simulink model "EMT_ML.before_diagnostic_fixes"  (R2024b)
settings: Solver=ode5  StartTime=0.0  StopTime=200  FixedStep=0.002  RelTol=1e-3
model workspace (MAT data in the model file):
  A = 7.3
  B = 2.71
  C0_shift = 200
  C1_shift = 200
  C2_shift = 200
  Cb = 70
  Cd = 0.6
  EMSInputBus : Simulink.Bus (value not decoded)
  Fb_max = 247500
  JA = 0.4
  JB = 0.4
  JZ = 0.4
  Jc1r2 = 0.01
  Jc3r4 = 0.01
  Jc4 = 0.01
  Je = 2.5
  Jh = 0.01
  Jq1 = 0.01
  Jq2 = 0.01
  Jr1 = 0.01
  Jr3s4 = 0.01
  Js123 = 0.01
  L = 4.472
  NE = [1600 1600 1600 1600 1600 1600 1600 1600 1600 1600 1600 1600 ... (840 elements, 30x28)]
  N_Te = 30
  N_ne = 28
  PE = [0 100.366530527 133.710336161 167.221698607 195.706356687 221.845219395 250.497434286 278.144308305 305.288511886 330.086920096 352.87464656 374.489475338 ... (840 elements, 30x28)]
  PN0 = 0
  Pb_epr = [-45 -45 -40 -30 0 30 40 45 45]
  Pb_max = [0 40 45 45 45]
  Pb_min = [-45 -45 -45 -40 0]
  Pe_ass = 230
  Pe_max = 1103
  Peg = [0 100 120 140 160 180 200 220 240 260 280 300 ... (53 elements, 1x53)]
  R_map = [0.09 0.089 0.09 0.091 0.092 0.093 0.094 0.095 0.096 0.097 0.098]
  SF_C0 = 1.5
  SF_C1 = 1.5
  SF_C2 = 1.5
  SF_Z1 = 1.5
  SF_Z2 = 1.5
  SF_ZD = 1.5
  SOC0 = 60
  SOC_epr = [30 31 50 59 60 61 70 79 80]
  SOC_map = [0 10 20 30 40 50 60 70 80 90 100]
  TA_max_map = [588.855 593.803361345 598.83559322 603.953846154 609.160344828 614.457391304 619.847368421 625.332743363 630.916071429 636.6 642.387272727 648.280733945 ... (115 elements, 1x115)]
  TA_min_map = [-588.855 -593.803361345 -598.83559322 -603.953846154 -609.160344828 -614.457391304 -619.847368421 -625.332743363 -630.916071429 -636.6 -642.387272727 -648.280733945 ... (115 elements, 1x115)]
  TAf = 0
  TB_max_map = [588.855 593.803361345 598.83559322 603.953846154 609.160344828 614.457391304 619.847368421 625.332743363 630.916071429 636.6 642.387272727 648.280733945 ... (115 elements, 1x115)]
  TB_min_map = [-588.855 -593.803361345 -598.83559322 -603.953846154 -609.160344828 -614.457391304 -619.847368421 -625.332743363 -630.916071429 -636.6 -642.387272727 -648.280733945 ... (115 elements, 1x115)]
  TBf = 0
  TE = [0 599 798 998 1168 1324 1495 1660 1822 1970 2106 2235 ... (840 elements, 30x28)]
  TS_A = 0.2
  TS_B = 0.2
  TS_C0 = 0.2
  TS_C1 = 0.2
  TS_C2 = 0.2
  TS_Z = 0.2
  TS_Z1 = 0.2
  TS_Z2 = 0.2
  TS_ZD = 0.2
  TZ_max_map = [537.13125 540.509433962 543.930379747 547.394904459 550.903846154 554.458064516 558.058441558 561.705882353 565.401315789 569.145695364 572.94 576.785234899 ... (131 elements, 1x131)]
  TZ_min_map = [-537.13125 -540.509433962 -543.930379747 -547.394904459 -550.903846154 -554.458064516 -558.058441558 -561.705882353 -565.401315789 -569.145695364 -572.94 -576.785234899 ... (131 elements, 1x131)]
  TZf = 0
  T_generator = [0 185 493.333333333 801.666666667 1110 1418.33333333 1726.66666667]
  T_motor = [0 185 493.333333333 801.666666667 1110 1418.33333333 1726.66666667]
  Te_map = [0 599 798 998 1168 1324 1495 1660 1822 1970 2106 2235 ... (30 elements, 1x30)]
  Te_max = 2754
  Te_max_map = [1168 1324 1495 1660 1822 1970 2106 2235 2355 2458 2543 2606 ... (28 elements, 1x28)]
  Te_start = 1600
  Tef = 100
  Teg = [0 596.8125 636.6 718.741935484 799.916230366 859.41 954.422788606 954.9 996.417391304 1078.98305085 1114.05 1169.26530612 ... (53 elements, 1x53)]
  Temax = 998
  Time = [0 0.1 0.2 0.3 0.4 0.5 0.6 0.7 0.8 0.9 1 1.1 ... (2001 elements, 1x2001)]
  Time_ele = [0 4 8 12 16 20 24 28 32 36 40 44 ... (401 elements, 1x401)]
  Time_fg = [0 2 4 6 8 10 12 14 16 18 20 22 ... (801 elements, 1x801)]
  Tmax_C0 = 2754
  Tmax_C1 = 3505.25455609
  Tmax_C2 = 3505.25455609
  Tmax_Z1 = 5584.80955498
  Tmax_Z2 = 16307.6439005
  Tmax_ZD = 3855.6
  Ts_e = 0.1
  Uoc_map = [814.5 917 933.25 945.75 958.25 969.25 978 985.25 993.25 1003.25 1050]
  V_Shift12 = 32
  V_Shift21 = 25
  V_Start = 10
  Voltage0 = 900
  Voltage_epr = [750 760 900 1000 1050]
  Y_engine = 0.955
  Yc = 0.98
  Yh = 0.96
  Yo = 0.92
  Yq = 0.94
  Z1_shift = 200
  Z2_shift = 200
  a11 = 1.54241568346
  a11_L = 1.54241568346
  a12 = -3.86074191629
  a12_L = 2.43173643789
  a21 = -1.04963112005
  a22 = 2.46948356808
  b11 = 0
  b11_L = 0
  b12 = 3.33
  b12_L = 7.8036
  b21 = 2.23571428571
  b22 = -2.13
  c11 = -0.648333656565
  c12 = 0
  c21 = -0.648333656565
  c22 = 0.680511182109
  controller_id = 1
  controller_name = 'Existing heuristic-grid EMS'
  cycle_grade = [0 0 0 0 0 0 0 0 0 0 0 0 ... (2001 elements, 1x2001)]
  cycle_road = [0.045 0.045 0.045 0.045 0.045 0.045 0.045 0.045 0.045 0.045 0.045 0.045 ... (2001 elements, 1x2001)]
  cycle_steering = [0 0 0 0 0 0 0 0 0 0 0 0 ... (2001 elements, 1x2001)]
  cycle_time = [0 0.1 0.2 0.3 0.4 0.5 0.6 0.7 0.8 0.9 1 1.1 ... (2001 elements, 1x2001)]
  d11 = -0.751666343435
  d12 = 0.3003003003
  d21 = -0.751666343435
  d22 = 0.319488817891
  e11 = -1.54241568346
  e12 = 0
  e21 = 1.04963112005
  e22 = -2.23571428571
  eff_generator = [0.8 0.8 0.79 0.79 0.76 0.74 0.72 0.8 0.85 0.88 0.85 0.8 ... (84 elements, 7x12)]
  eff_motor = [0.8 0.8 0.79 0.79 0.76 0.74 0.72 0.8 0.85 0.88 0.85 0.8 ... (84 elements, 7x12)]
  ele_map = [10 11.46 14.13 19.24 20.94 23.21 20.29 20.23 22.28 17.66 16.24 18.95 ... (401 elements, 1x401)]
  ems_runtime_config : object (value not decoded)
  f11 = -3.86074191629
  f12 = 3.33
  f21 = 2.46948356808
  f22 = -2.13
  fg = 0.045
  fg_map = [0.0125 0.0215 0.0332 0.0452 0.0525 0.0589 0.0584 0.0592 0.0621 0.0576 0.055 0.0572 ... (801 elements, 1x801)]
  fuel_gpkwh = [269.874826377 269.874826377 260.084605263 254.895150301 249.802821062 244.062054381 234.972466555 226.630558735 223.93243551 227.612775381 231.379615385 228.983738255 ... (840 elements, 30x28)]
  fuel_map = [269.874826377 269.874826377 260.084605263 254.895150301 249.802821062 244.062054381 234.972466555 226.630558735 223.93243551 227.612775381 231.379615385 228.983738255 ... (840 elements, 30x28)]
  fuel_map_N = [269.874826377 269.874826377 260.084605263 254.895150301 249.802821062 nan nan nan nan nan nan nan ... (840 elements, 30x28)]
  i = 28
  ic = 4.42
  iq = 1.4
  it = 4
  j = 30
  k1 = 2.13
  k2 = 2.13
  k3 = 2.33
  k4 = 1.92
  kh = 2.88
  kq = 2.17
  kt = 1.83
  mass = 45000
  miu_max = 0.8
  nA_map = [-6000 -5950 -5900 -5850 -5800 -5750 -5700 -5650 -5600 -5550 -5500 -5450 ... (115 elements, 1x115)]
  nA_max = 6000
  nA_min = -6000
  nB_map = [-6000 -5950 -5900 -5850 -5800 -5750 -5700 -5650 -5600 -5550 -5500 -5450 ... (115 elements, 1x115)]
  nB_max = 6000
  nB_min = -6000
  nB_start = 0
  nZ_map = [-8000 -7950 -7900 -7850 -7800 -7750 -7700 -7650 -7600 -7550 -7500 -7450 ... (131 elements, 1x131)]
  nZ_max = 8000
  nZ_min = -8000
  n_generator = [0 318.5 796.25 1274 1751.75 2229.5 2707.25 3185 3662.75 4140.5 4618.25 7007]
  n_motor = [0 318.5 796.25 1274 1751.75 2229.5 2707.25 3185 3662.75 4140.5 4618.25 7007]
  ne_idl = 3000
  ne_map = [1600 1700 1800 1900 2000 2100 2200 2300 2400 2500 2600 2700 ... (28 elements, 1x28)]
  ne_max = 4200
  ne_min = 1600
  ne_start = 200
  neg = [1600 1600 1800 1860 1910 2000 2001 2200 2300 2301 2400 2450 ... (53 elements, 1x53)]
  no_Shift12 = 1589.43589002
  no_Shift21 = 1241.74678908
  rz = 0.318
  startup_feedback_delay_s = 0.002
  startup_power_share = 0.5
  startup_speed_regularizer_rpm = 100
  v_cyc = [0 0 0 0 0 0 0 0 0 0 0 0 ... (2001 elements, 1x2001)]
  voltage_HighA = 1050
  voltage_HighB = 1050
  voltage_HighZ = 1050
  voltage_LowA = 750
  voltage_LowB = 750
  voltage_LowZ = 750
symbols that are objects in the model workspace (value not decoded): ems_runtime_config
undefined symbols (not defined in the file or in its folder): sigbuilder_block
libraries: fl_lib x82, nesl_utility x55, simulink x49, sdl_lib x10, simulink_need_slupdate x6, powerlib_extras x1
(part 4 of 7)

== system EMT_ML.before_diagnostic_fixes/Control Unit/Control/Power Distribution/Electric Power Requirement ==
  Voltage : Inport
  SOC : Inport  Port=2
  ElectricPower : Inport  Port=3
  1-D Lookup Table : Lookup_n-D  NumberOfTableDimensions=1  BreakpointsForDimension1=SOC_epr  Table=Pb_epr  RndMeth=Simplest
  1-D Lookup Table2 : Lookup_n-D  NumberOfTableDimensions=1  BreakpointsForDimension1=Voltage_epr  Table=Pb_max  RndMeth=Simplest
  1-D Lookup Table3 : Lookup_n-D  NumberOfTableDimensions=1  BreakpointsForDimension1=Voltage_epr  Table=Pb_min  RndMeth=Simplest
  Add : Sum  Inputs=+--
  Constant : Constant  Value=PN0
  Data : Subsystem
  Memory3 : Memory  InitialCondition=SOC0
  Memory7 : Memory  InitialCondition=SOC0
  Mux : Mux
  PZ_com : Constant  Value=0
  Saturation1 : Saturate  UpperLimit=max(SOC_epr)  LowerLimit=min(SOC_epr)
  Saturation2 : Saturate  UpperLimit=max(Voltage_epr)  LowerLimit=min(Voltage_epr)
  PN_k : Outport
  wires:
  1-D Lookup Table2/1 -> Data/2(PN_max), Mux/2
  1-D Lookup Table3/1 -> Data/3(PN_min), Mux/3
  Saturation2/1 -> 1-D Lookup Table3/1, 1-D Lookup Table2/1
  Voltage/1 -> Memory7/1
  Saturation1/1 -> 1-D Lookup Table/1
  Add/1 -> Data/1(PN_com), Mux/1
  1-D Lookup Table/1 -> Add/1
  Memory3/1 -> Saturation1/1
  SOC/1 -> Memory3/1
  Mux/1 -> PN_k/1
  Memory7/1 -> Saturation2/1
  Constant/1 -> Add/3
  ElectricPower/1 -> Add/2
  PZ_com/1 -> Mux/4

== system EMT_ML.before_diagnostic_fixes/Control Unit/Control/Power Distribution/Feasible Control Range ==
  stage : Inport
  ne_act : Inport  Port=2
  v_act : Inport  Port=3
  Memory1 : Memory
  Memory5 : Memory
  State Calculation : Subsystem
  State Predition : Subsystem
  stage_k : Outport
  ne_k : Outport  Port=2
  no_k : Outport  Port=3
  Te_k : Outport  Port=4
  TA_k : Outport  Port=5
  TB_k : Outport  Port=6
  wires:
  State Predition/3(no_k) -> no_k/1
  State Predition/4(Te_k) -> Te_k/1
  State Predition/5(TA_k) -> TA_k/1
  State Predition/6(TB_k) -> TB_k/1
  State Predition/2(ne_k) -> ne_k/1
  State Predition/1(stage_k) -> stage_k/1
  ne_act/1 -> Memory5/1
  stage/1 -> State Calculation/1(s)
  v_act/1 -> Memory1/1
  Memory5/1 -> State Calculation/2(ne)
  Memory1/1 -> State Calculation/3(v_act)
  State Calculation/1(stage) -> State Predition/1(stage)
  State Calculation/2(ne_act) -> State Predition/2(ne_act)
  State Calculation/3(nA_act) -> State Predition/3(nA_act)
  State Calculation/4(nB_act) -> State Predition/4(nB_act)
  State Calculation/5(no_act) -> State Predition/5(no_act)

== system EMT_ML.before_diagnostic_fixes/Control Unit/Control/Power Distribution/Oil Control ==
  Demux : Demux
      settings: DisplayOption=none
  Transfer Fcn1 : TransferFcn  Denominator=[TS_C0 1]
  Transfer Fcn2 : TransferFcn  Denominator=[TS_Z1 1]
  Transfer Fcn3 : TransferFcn  Denominator=[TS_Z2 1]
  Transfer Fcn4 : TransferFcn  Denominator=[TS_C1 1]
  tag scope: Press_C0=global, Press_C1=global, Press_Z1=global, Press_Z2=global
  wires:
  Transfer Fcn1/1 -> [Press_C0]
  Transfer Fcn2/1 -> [Press_Z1]
  Demux/1 -> Transfer Fcn1/1
  Demux/4 -> Transfer Fcn4/1
  Demux/3 -> Transfer Fcn3/1
  Demux/2 -> Transfer Fcn2/1
  Transfer Fcn4/1 -> [Press_C1]
  Transfer Fcn3/1 -> [Press_Z2]
  [Press] -> Demux/1

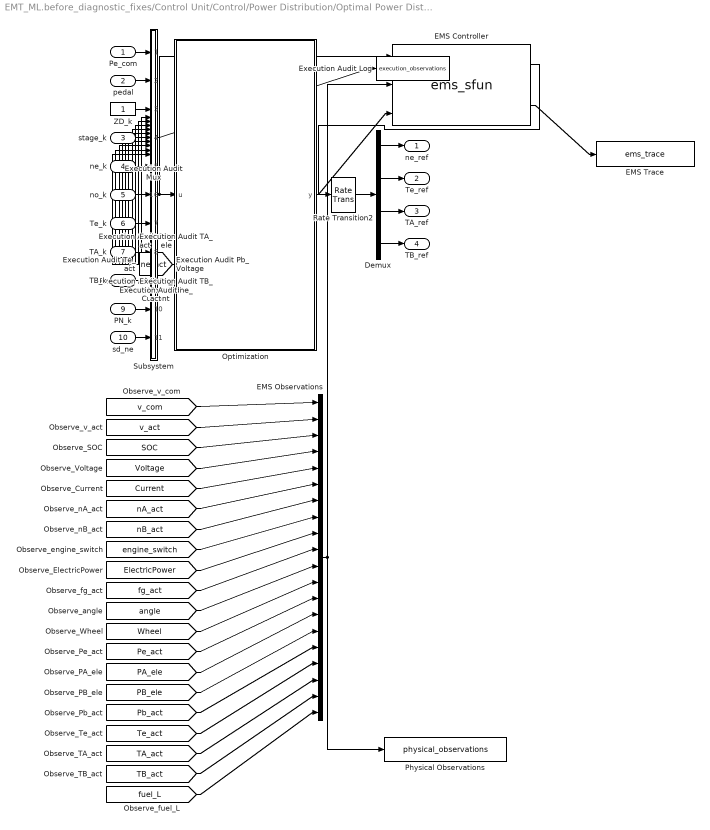
== system EMT_ML.before_diagnostic_fixes/Control Unit/Control/Power Distribution/Optimal Power Distribution ==
  Pe_com : Inport
  pedal : Inport  Port=2
  stage_k : Inport  Port=3
  ne_k : Inport  Port=4
  no_k : Inport  Port=5
  Te_k : Inport  Port=6
  TA_k : Inport  Port=7
  TB_k : Inport  Port=8
  PN_k : Inport  Port=9
  sd_ne : Inport  Port=10
  Demux : Demux
  EMS Controller : M-S-Function  FunctionName=ems_sfun  Parameters=ems_runtime_config,controller_id
  EMS Observations : Mux  Inputs=20
  EMS Trace : ToWorkspace  VariableName=ems_trace  SaveFormat=Structure With Time  SampleTime=0.02
  Execution Audit Log : ToWorkspace  VariableName=execution_observations  SaveFormat=Structure With Time  SampleTime=0.002
  Execution Audit Mux : Mux  Inputs=10
  "Optimization " : MATLAB Function  TreatAsAtomicUnit=on  SystemSampleTime=0.02
  Physical Observations : ToWorkspace  VariableName=physical_observations  SaveFormat=Structure With Time  SampleTime=0.002
  Rate Transition2 : RateTransition
  Subsystem : Subsystem  mask{Parameter1=on}
      mask prompts: Parameter1 "11"
  ZD_k : Constant
  ne_ref : Outport
  Te_ref : Outport  Port=2
  TA_ref : Outport  Port=3
  TB_ref : Outport  Port=4
  wires:
  Demux/1 -> ne_ref/1
  pedal/1 -> Subsystem/2(In2)
  Pe_com/1 -> Subsystem/1(In1)
  ZD_k/1 -> Subsystem/3(In3)
  ne_k/1 -> Subsystem/5(In5)
  no_k/1 -> Subsystem/6(In6)
  Te_k/1 -> Subsystem/7(In7)
  TA_k/1 -> Subsystem/8(In8)
  TB_k/1 -> Subsystem/9(In9)
  PN_k/1 -> Subsystem/10(In10)
  Demux/4 -> TB_ref/1
  Demux/3 -> TA_ref/1
  Demux/2 -> Te_ref/1
  Subsystem/1(Out) -> "Optimization "/1(u), EMS Controller/1
  stage_k/1 -> Subsystem/4(In4)
  Rate Transition2/1 -> Demux/1
  sd_ne/1 -> Subsystem/11(In11)
  [v_com] -> EMS Observations/1
  [v_act] -> EMS Observations/2
  [SOC] -> EMS Observations/3
  [Voltage] -> EMS Observations/4
  [Current] -> EMS Observations/5
  [nA_act] -> EMS Observations/6
  [nB_act] -> EMS Observations/7
  [engine_switch] -> EMS Observations/8
  [ElectricPower] -> EMS Observations/9
  [fg_act] -> EMS Observations/10
  [angle] -> EMS Observations/11
  [Wheel] -> EMS Observations/12
  [Pe_act] -> EMS Observations/13
  [PA_ele] -> EMS Observations/14
  [PB_ele] -> EMS Observations/15
  [Pb_act] -> EMS Observations/16
  [Te_act] -> EMS Observations/17
  [TA_act] -> EMS Observations/18
  [TB_act] -> EMS Observations/19
  [fuel_L] -> EMS Observations/20
  EMS Observations/1 -> EMS Controller/2, Physical Observations/1
  "Optimization "/1(y) -> EMS Controller/3
  EMS Controller/1 -> Rate Transition2/1
  EMS Controller/2 -> EMS Trace/1
  [ne_act] -> Execution Audit Mux/1
  [Te_act] -> Execution Audit Mux/2
  [Pe_act] -> Execution Audit Mux/3
  [TA_act] -> Execution Audit Mux/4
  [TB_act] -> Execution Audit Mux/5
  [PA_ele] -> Execution Audit Mux/6
  [PB_ele] -> Execution Audit Mux/7
  [Pb_act] -> Execution Audit Mux/8
  [Current] -> Execution Audit Mux/9
  [Voltage] -> Execution Audit Mux/10
  Execution Audit Mux/1 -> Execution Audit Log/1

== system EMT_ML.before_diagnostic_fixes/Control Unit/Control/Power Distribution/Pedal Interpretation ==
  Pedal : Inport
  Brake Control : Subsystem
  Data : Subsystem
  Engine Power Requirement : Subsystem
  Subsystem7 : Subsystem
  Subsystem8 : Subsystem
  Fb_ref : Outport
  Pe_com : Outport  Port=2
  wires:
  Engine Power Requirement/1(Pe_com) -> Pe_com/1, Data/3(Pe_com)
  Pedal/1 -> Subsystem7/1(0), Subsystem8/1(0)
  Subsystem7/1(1) -> Engine Power Requirement/1(Acc_pedal), Data/2(Acc_pedal)
  Subsystem8/1(1) -> Brake Control/1(Dec_pedal), Data/1(Dec_pedal)
  Brake Control/1(Fb_ref) -> Fb_ref/1

== system EMT_ML.before_diagnostic_fixes/Control Unit/Control/Power Distribution/Subsystem ==
  Discrete PID Controller : powerlib_extras/Discrete  Control Blocks/Discrete PID Controller  Kp=0.5  Ki=0.1  Kd=0  TcD=1  Par_Limits=[200 -200]  Init=0  Ts=0.5
  Sum : Sum  Inputs=|+-
  sd_ne : Outport
  wires:
  [ne_act] -> Sum/2
  Sum/1 -> Discrete PID Controller/1
  Discrete PID Controller/1 -> sd_ne/1
  [ne_ref] -> Sum/1

== system EMT_ML.before_diagnostic_fixes/Control Unit/Control/Prepare Stage/brack force ==
  Constant1 : Constant  Value=Fb_max
  Fb_com : Outport
  wires:
  Constant1/1 -> Fb_com/1

== system EMT_ML.before_diagnostic_fixes/Control Unit/Control/Prepare Stage/clutches condition ==
  Mux1 : Mux
  Subsystem : Subsystem
  Subsystem1 : Subsystem
  Subsystem2 : Subsystem
  Subsystem3 : Subsystem
  clutch_com : Outport
  wires:
  Subsystem/1(C0) -> Mux1/1
  Subsystem2/1(C1) -> Mux1/4
  Subsystem1/1(Z2) -> Mux1/3
  Subsystem3/1(Z1) -> Mux1/2
  Mux1/1 -> clutch_com/1

== system EMT_ML.before_diagnostic_fixes/Control Unit/Control/Prepare Stage/engine swich ==
  Compare To Constant2 : simulink/Logic and Bit Operations/Compare To Constant  relop=>  const=ne_start  OutDataTypeStr=uint8
  Constant : Constant
  Memory2 : Memory
  Triggered Subsystem : Subsystem  TreatAsAtomicUnit=on
  engine_swich : Outport
  wires:
  Triggered Subsystem/1(Out1) -> engine_swich/1
  Constant/1 -> Triggered Subsystem/1(In1)
  Memory2/1 -> Compare To Constant2/1
  [ne_act] -> Memory2/1
  Compare To Constant2/1 -> Triggered Subsystem/Trigger

== system EMT_ML.before_diagnostic_fixes/Control Unit/Control/Prepare Stage/engine torque ==
  Subsystem1 : Subsystem
  Te_com : Outport
  wires:
  Subsystem1/1(Te_com) -> Te_com/1
  [ne_act] -> Subsystem1/1(ne_act)

== system EMT_ML.before_diagnostic_fixes/Control Unit/Control/Prepare Stage/motorA torque ==
  Constant2 : Constant  Value=0
  Subsystem : Subsystem
  Switch : Switch  Criteria=u2 > Threshold  Threshold=0.1  SaturateOnIntegerOverflow=off  InputSameDT=off
  TA_com1 : Subsystem
  TA_com : Outport
  wires:
  Switch/1 -> TA_com/1
  Subsystem/1(Judge) -> Switch/2
  Constant2/1 -> Switch/3
  TA_com1/1(TA_com) -> Switch/1

== system EMT_ML.before_diagnostic_fixes/Control Unit/Control/Prepare Stage/motorB torque ==
  Lookup Table : Lookup  InputValues=nB_map  Table=TB_max_map*1.5  SaturateOnIntegerOverflow=off
  Lookup Table1 : Lookup  InputValues=nB_map  Table=TB_min_map*1.5  SaturateOnIntegerOverflow=off
  Saturation Dynamic : simulink/Discontinuities/Saturation Dynamic  OutMin=[]  OutMax=[]  OutDataTypeStr=Inherit: Same as second input  OutDataType=sfix(16)  OutScaling=2^-10  DoSatur=off
  Saturation1 : Saturate  UpperLimit=max(nB_map)  LowerLimit=min(nB_map)
  Saturation2 : Saturate  UpperLimit=max(nB_map)  LowerLimit=min(nB_map)
  Subsystem1 : Subsystem
  TB_com : Outport
  wires:
  Saturation Dynamic/1 -> TB_com/1
  [nB_act] -> Subsystem1/1(nB_act), Saturation1/1, Saturation2/1
  Lookup Table/1 -> Saturation Dynamic/1
  Lookup Table1/1 -> Saturation Dynamic/3
  Saturation1/1 -> Lookup Table/1
  Saturation2/1 -> Lookup Table1/1
  Subsystem1/1(TB_com) -> Saturation Dynamic/2

== system EMT_ML.before_diagnostic_fixes/Control Unit/Control/Prepare Stage/motorZ torque ==
  Lookup Table : Lookup  InputValues=nZ_map  Table=TZ_max_map  SaturateOnIntegerOverflow=off
  Lookup Table1 : Lookup  InputValues=nZ_map  Table=TZ_min_map  SaturateOnIntegerOverflow=off
  Saturation Dynamic : simulink/Discontinuities/Saturation Dynamic  OutMin=[]  OutMax=[]  OutDataTypeStr=Inherit: Same as second input  OutDataType=sfix(16)  OutScaling=2^-10  DoSatur=off
  Saturation1 : Saturate  UpperLimit=max(nZ_map)  LowerLimit=min(nZ_map)
  Saturation2 : Saturate  UpperLimit=max(nZ_map)  LowerLimit=min(nZ_map)
  Subsystem1 : Subsystem
  TZ_com : Outport
  wires:
  Saturation Dynamic/1 -> TZ_com/1
  [nZ_act] -> Saturation1/1, Saturation2/1, Subsystem1/1(nZ_act)
  Lookup Table/1 -> Saturation Dynamic/1
  Lookup Table1/1 -> Saturation Dynamic/3
  Saturation1/1 -> Lookup Table/1
  Saturation2/1 -> Lookup Table1/1
  Subsystem1/1(TZ_com) -> Saturation Dynamic/2

== system EMT_ML.before_diagnostic_fixes/Control Unit/Control/Shift Stage/EVT1->EVT2 ==
  Mux : Mux  Inputs=7
  brack force : Subsystem
  clutches condition : Subsystem
  engine swich : Subsystem
  engine torque : Subsystem
  motorA torque : Subsystem
  motorB torque : Subsystem
  motorZ torque : Subsystem
  control : Outport
  wires:
  motorB torque/1(TB_com) -> Mux/5
  motorA torque/1(TA_com) -> Mux/4
  engine torque/1(Te_com) -> Mux/3
  Mux/1 -> control/1
  engine swich/1(engine_swich) -> Mux/2
  clutches condition/1(clutch_com) -> Mux/1
  brack force/1(Fb_com) -> Mux/7
  motorZ torque/1(TZ_com) -> Mux/6

== system EMT_ML.before_diagnostic_fixes/Control Unit/Control/Shift Stage/EVT2->EVT1 ==
  Mux : Mux  Inputs=7
  brack force : Subsystem
  clutches condition : Subsystem
  engine swich : Subsystem
  engine torque : Subsystem
  motorA torque : Subsystem
  motorB torque : Subsystem
  motorZ torque : Subsystem
  control : Outport
  wires:
  motorB torque/1(TB_com) -> Mux/5
  motorA torque/1(TA_com) -> Mux/4
  Mux/1 -> control/1
  engine torque/1(Te_com) -> Mux/3
  engine swich/1(engine_swich) -> Mux/2
  clutches condition/1(clutch_com) -> Mux/1
  brack force/1(Fb_com) -> Mux/7
  motorZ torque/1(TZ_com) -> Mux/6

== system EMT_ML.before_diagnostic_fixes/Control Unit/Control/Shift Stage/Shift Judge ==
  1 : Constant
  Add : Sum
  Compare To Constant1 : simulink/Logic and Bit Operations/Compare To Constant  relop=>  const=1  OutDataTypeStr=uint8
  Data Type Conversion1 : DataTypeConversion  SaturateOnIntegerOverflow=off  RndMeth=Floor
  Fcn : Fcn  Expr=V_Shift21+5*u
  Logical Operator1 : Logic  AllPortsSameDT=off  OutDataTypeStr=boolean
  Memory1 : Memory
  Memory2 : Memory
  Memory5 : Memory
  Relational Operator : RelationalOperator  Operator=<=  OutDataTypeStr=boolean  InputSameDT=off
  shift : Outport
  wires:
  Data Type Conversion1/1 -> Add/2
  Fcn/1 -> Relational Operator/2
  Memory1/1 -> Fcn/1
  [Acc_pedal] -> Memory1/1
  Logical Operator1/1 -> Data Type Conversion1/1
  Compare To Constant1/1 -> Logical Operator1/2
  Relational Operator/1 -> Logical Operator1/1
  [v_act] -> Memory2/1
  Memory2/1 -> Relational Operator/1
  [stage] -> Memory5/1
  Memory5/1 -> Compare To Constant1/1
  1/1 -> Add/1
  Add/1 -> shift/1

== system EMT_ML.before_diagnostic_fixes/Control Unit/Control/Stage Judge/EVT1_H Stage ==
  Compare To Constant1 : simulink/Logic and Bit Operations/Compare To Constant  relop=>  const=0.9  OutDataTypeStr=uint8
  Compare To Constant6 : simulink/Logic and Bit Operations/Compare To Constant  relop=>=  const=0.9  OutDataTypeStr=uint8
  Data Type Conversion : DataTypeConversion  SaturateOnIntegerOverflow=off  RndMeth=Floor
  Logical Operator1 : Logic  AllPortsSameDT=off  OutDataTypeStr=boolean
  Memory1 : Memory
  Memory6 : Memory
  Out1 : Outport
  wires:
  Data Type Conversion/1 -> Out1/1
  Logical Operator1/1 -> Data Type Conversion/1
  Memory1/1 -> Compare To Constant1/1
  [Press_C0] -> Memory1/1
  [Press_Z2] -> Memory6/1
  Memory6/1 -> Compare To Constant6/1
  Compare To Constant1/1 -> Logical Operator1/1
  Compare To Constant6/1 -> Logical Operator1/2

== system EMT_ML.before_diagnostic_fixes/Control Unit/Control/Stage Judge/EVT2 Stage ==
  Add : Sum
  Compare To Constant10 : simulink/Logic and Bit Operations/Compare To Constant  relop=>=  const=2  OutDataTypeStr=uint8
  Compare To Constant11 : simulink/Logic and Bit Operations/Compare To Constant  relop=>  const=0.1  OutDataTypeStr=uint8
  Compare To Constant2 : simulink/Logic and Bit Operations/Compare To Constant  relop=<  const=0.9  OutDataTypeStr=uint8
  Compare To Constant3 : simulink/Logic and Bit Operations/Compare To Constant  relop=<=  const=0.1  OutDataTypeStr=uint8
  Compare To Constant4 : simulink/Logic and Bit Operations/Compare To Constant  relop=>=  const=0.9  OutDataTypeStr=uint8
  Data Type Conversion : DataTypeConversion  SaturateOnIntegerOverflow=off  RndMeth=Floor
  Gain : Gain  Gain=3
  Gain1 : Gain  Gain=2
  Logical Operator : Logic  AllPortsSameDT=off  OutDataTypeStr=boolean
  Logical Operator4 : Logic  Inputs=3  AllPortsSameDT=off  OutDataTypeStr=boolean
  Memory{2..4,10..11} (5 alike) : Memory
  Out1 : Outport
  wires:
  Gain1/1 -> Add/1
  Data Type Conversion/1 -> Out1/1
  Add/1 -> Data Type Conversion/1
  Logical Operator4/1 -> Gain1/1
  Gain/1 -> Add/2
  [Press_Z2] -> Memory3/1
  Memory3/1 -> Compare To Constant3/1
  [Press_C1] -> Memory4/1
  Memory4/1 -> Compare To Constant4/1
  Compare To Constant3/1 -> Logical Operator/1
  Compare To Constant4/1 -> Logical Operator/2
  Logical Operator/1 -> Gain/1
  Compare To Constant2/1 -> Logical Operator4/2
  [Press_Z2] -> Memory2/1
  Memory2/1 -> Compare To Constant2/1
  [stage] -> Memory10/1
  Memory10/1 -> Compare To Constant10/1
  Compare To Constant10/1 -> Logical Operator4/1
  [Press_Z2] -> Memory11/1
  Memory11/1 -> Compare To Constant11/1
  Compare To Constant11/1 -> Logical Operator4/3

== system EMT_ML.before_diagnostic_fixes/Control Unit/Control/Stage Judge/Prepare Stage ==
  Constant2 : Constant  Value=0
  Out1 : Outport
  wires:
  Constant2/1 -> Out1/1

== system EMT_ML.before_diagnostic_fixes/Control Unit/Control/Stage Judge/Shift Stage ==
  Compare To Constant5 : simulink/Logic and Bit Operations/Compare To Constant  relop=>  const=0.1  OutDataTypeStr=uint8
  Compare To Constant9 : simulink/Logic and Bit Operations/Compare To Constant  relop=>  const=0.1  OutDataTypeStr=uint8
  Data Type Conversion : DataTypeConversion  SaturateOnIntegerOverflow=off  RndMeth=Floor
  Logical Operator2 : Logic  AllPortsSameDT=off  OutDataTypeStr=boolean
  Memory5 : Memory
  Memory9 : Memory
  Out1 : Outport
  wires:
  Data Type Conversion/1 -> Out1/1
  Logical Operator2/1 -> Data Type Conversion/1
  Compare To Constant5/1 -> Logical Operator2/2
  [Press_C1] -> Memory5/1
  Memory5/1 -> Compare To Constant5/1
  [Press_Z2] -> Memory9/1
  Memory9/1 -> Compare To Constant9/1
  Compare To Constant9/1 -> Logical Operator2/1

== system EMT_ML.before_diagnostic_fixes/Control Unit/Driver/Electric Power Requirement/Subsystem4 ==
  Subsystem4 : Subsystem
  Subsystem6 : Subsystem
  Out1 : Outport
  Out2 : Outport  Port=2
  Out3 : Outport  Port=3
  Out4 : Outport  Port=4
  Out5 : Outport  Port=5
  Out6 : Outport  Port=6
  Out7 : Outport  Port=7
  Out8 : Outport  Port=8
  wires:
  Subsystem4/4(100) -> Out8/1
  Subsystem4/3(10) -> Out7/1
  Subsystem4/2(0.01) -> Out6/1
  Subsystem4/1(0.1) -> Out5/1
  Subsystem6/4(4) -> Out4/1
  Subsystem6/3(3) -> Out3/1
  Subsystem6/2(2) -> Out2/1
  Subsystem6/1(1) -> Out1/1

== system EMT_ML.before_diagnostic_fixes/Control Unit/Driver/Electric Power Requirement/Subsystem6 ==
  Add : Inport
  Sub : Inport  Port=2
  0.1 : Inport  Port=3
  10 : Inport  Port=4
  0.2 : InportShadow  Port=3
  1 : InportShadow  Port=4
  Add1 : Sum  Inputs=++-
  Memory1 : Memory
  Saturation : Saturate  UpperLimit=800  LowerLimit=0
  Subsystem : Subsystem
  Subsystem1 : Subsystem
  Transfer Fcn2 : TransferFcn  Denominator=[0.05 1]
  Power : Outport
  wires:
  Add1/1 -> Memory1/1, Saturation/1
  Memory1/1 -> Add1/1
  Subsystem1/1(power--) -> Add1/3
  Saturation/1 -> Transfer Fcn2/1
  Subsystem/1(power++) -> Add1/2
  0.1/1 -> Subsystem/1(0.1)
  Add/1 -> Subsystem/2(Add)
  10/1 -> Subsystem/3(10)
  Sub/1 -> Subsystem1/2(Sub)
  1/1 -> Subsystem1/3(10)
  0.2/1 -> Subsystem1/1(0.1)
  Transfer Fcn2/1 -> Power/1

== system EMT_ML.before_diagnostic_fixes/Control Unit/Driver/Gears/Subsystem ==
  Add : Inport
  Sub : Inport  Port=2
  Add1 : Sum  Inputs=++-
  Data Type Conversion : DataTypeConversion  SaturateOnIntegerOverflow=off  RndMeth=Floor
  Data Type Conversion1 : DataTypeConversion  SaturateOnIntegerOverflow=off  RndMeth=Floor
  Memory1 : Memory  InitialCondition=1
  Memory2 : Memory
  Memory3 : Memory
  Relational Operator : RelationalOperator  Operator=~=  OutDataTypeStr=boolean  InputSameDT=off
  Relational Operator1 : RelationalOperator  Operator=~=  OutDataTypeStr=boolean  InputSameDT=off
  Saturation : Saturate  UpperLimit=4  LowerLimit=0
  Gear : Outport
  wires:
  Add1/1 -> Memory1/1, Saturation/1
  Memory1/1 -> Add1/1
  Memory2/1 -> Relational Operator/2
  Add/1 -> Relational Operator/1, Memory2/1
  Memory3/1 -> Relational Operator1/2
  Sub/1 -> Relational Operator1/1, Memory3/1
  Relational Operator1/1 -> Data Type Conversion/1
  Relational Operator/1 -> Data Type Conversion1/1
  Data Type Conversion/1 -> Add1/3
  Data Type Conversion1/1 -> Add1/2
  Saturation/1 -> Gear/1

== system EMT_ML.before_diagnostic_fixes/Control Unit/Driver/Gears/Subsystem1 ==
  11 : Constant
  21 : Constant  Value=2
  22 : Constant  Value=3
  31 : Constant  Value=4
  1 : Outport
  2 : Outport  Port=2
  3 : Outport  Port=3
  4 : Outport  Port=4
  wires:
  11/1 -> 1/1
  21/1 -> 2/1
  22/1 -> 3/1
  31/1 -> 4/1

== system EMT_ML.before_diagnostic_fixes/Control Unit/Driver/Grade Angle/Subsystem4 ==
  Subsystem4 : Subsystem
  Subsystem6 : Subsystem
  Out1 : Outport
  Out2 : Outport  Port=2
  Out3 : Outport  Port=3
  Out4 : Outport  Port=4
  Out5 : Outport  Port=5
  Out6 : Outport  Port=6
  Out7 : Outport  Port=7
  Out8 : Outport  Port=8
  wires:
  Subsystem4/4(100) -> Out8/1
  Subsystem4/3(10) -> Out7/1
  Subsystem4/2(0.01) -> Out6/1
  Subsystem4/1(0.1) -> Out5/1
  Subsystem6/4(4) -> Out4/1
  Subsystem6/3(3) -> Out3/1
  Subsystem6/2(2) -> Out2/1
  Subsystem6/1(1) -> Out1/1

== system EMT_ML.before_diagnostic_fixes/Control Unit/Driver/Grade Angle/Subsystem6 ==
  Add : Inport
  Sub : Inport  Port=2
  0.1 : Inport  Port=3
  10 : Inport  Port=4
  0.2 : InportShadow  Port=3
  1 : InportShadow  Port=4
  Add1 : Sum  Inputs=++-
  Memory1 : Memory
  Saturation : Saturate  UpperLimit=40  LowerLimit=-40
  Subsystem : Subsystem
  Subsystem1 : Subsystem
  Transfer Fcn1 : TransferFcn  Denominator=[0.02 1]
  angle : Outport
  wires:
  Add1/1 -> Memory1/1, Saturation/1
  Memory1/1 -> Add1/1
  Subsystem1/1(angle-) -> Add1/3
  Saturation/1 -> Transfer Fcn1/1
  Subsystem/1(angle++) -> Add1/2
  0.1/1 -> Subsystem/1(0.1)
  Add/1 -> Subsystem/2(Add)
  10/1 -> Subsystem/3(10)
  Sub/1 -> Subsystem1/2(Sub)
  1/1 -> Subsystem1/3(10)
  0.2/1 -> Subsystem1/1(0.1)
  Transfer Fcn1/1 -> angle/1

== system EMT_ML.before_diagnostic_fixes/Control Unit/Driver/Ground Resistance Coefficient/Road ==
  Memory1 : Memory
  Multiport Switch : MultiPortSwitch  DataPortOrder=Zero-based contiguous  Inputs=4  zeroidx=on  SaturateOnIntegerOverflow=off  InputSameDT=off
  Subsystem : Subsystem
  Subsystem1 : Subsystem
  Subsystem2 : Subsystem
  Subsystem3 : Subsystem
  Subsystem4 : Subsystem
  fg : Outport
  wires:
  Memory1/1 -> Subsystem2/1(In1), Subsystem/1(In)
  Subsystem3/1(Out1) -> Multiport Switch/4
  Subsystem2/1(Out1) -> Multiport Switch/3
  Subsystem1/1(Out1) -> Multiport Switch/2
  Subsystem/1(Judge) -> Multiport Switch/1
  Subsystem4/1(Out1) -> Multiport Switch/5
  Multiport Switch/1 -> fg/1
  [Pedal] -> Memory1/1

== system EMT_ML.before_diagnostic_fixes/Control Unit/Driver/Ground Resistance Coefficient/Road1 ==
  1-D Lookup Table : Lookup_n-D  NumberOfTableDimensions=1  BreakpointsForDimension1=[-1 0 0.8 0.9 1]  Table=[10 5 2 1 0.8]  RndMeth=Simplest
  1-D Lookup Table1 : Lookup_n-D  NumberOfTableDimensions=1  BreakpointsForDimension1=[0 10 30 50 60 70 80 90]  Table=[0.16 0.16 0.12 0.10 0.08 0.06 0.05 0.05]  RndMeth=Simplest
  Memory1 : Memory
  Memory2 : Memory
  Product : Product  RndMeth=Zero
  fg : Outport
  wires:
  [Pedal] -> Memory1/1
  [v_act] -> Memory2/1
  Memory2/1 -> 1-D Lookup Table1/1
  Memory1/1 -> 1-D Lookup Table/1
  1-D Lookup Table/1 -> Product/1
  1-D Lookup Table1/1 -> Product/2
  Product/1 -> fg/1

== system EMT_ML.before_diagnostic_fixes/Control Unit/Driver/Ground Resistance Coefficient/Subsystem2 ==
  Subsystem4 : Subsystem
  Subsystem6 : Subsystem
  Out1 : Outport
  Out2 : Outport  Port=2
  Out3 : Outport  Port=3
  Out4 : Outport  Port=4
  Out5 : Outport  Port=5
  Out6 : Outport  Port=6
  Out7 : Outport  Port=7
  Out8 : Outport  Port=8
  wires:
  Subsystem6/1(1) -> Out1/1
  Subsystem6/2(2) -> Out2/1
  Subsystem6/3(3) -> Out3/1
  Subsystem6/4(4) -> Out4/1
  Subsystem4/1(0.1) -> Out5/1
  Subsystem4/2(0.01) -> Out6/1
  Subsystem4/3(10) -> Out7/1
  Subsystem4/4(100) -> Out8/1

== system EMT_ML.before_diagnostic_fixes/Control Unit/Driver/Ground Resistance Coefficient/Subsystem3 ==
  Add : Inport
  Sub : Inport  Port=2
  0.1 : Inport  Port=3
  10 : Inport  Port=4
  0.2 : InportShadow  Port=3
  1 : InportShadow  Port=4
  Add1 : Sum  Inputs=++-
  Memory1 : Memory  InitialCondition=0.04
  Subsystem : Subsystem
  Subsystem1 : Subsystem
  fg : Outport
  wires:
  0.2/1 -> Subsystem1/1(0.1)
  1/1 -> Subsystem1/3(10)
  Sub/1 -> Subsystem1/2(Sub)
  10/1 -> Subsystem/3(10)
  Add/1 -> Subsystem/2(Add)
  0.1/1 -> Subsystem/1(0.1)
  Subsystem/1(fg++) -> Add1/2
  Subsystem1/1(fg--) -> Add1/3
  Memory1/1 -> Add1/1
  Add1/1 -> fg/1, Memory1/1

== system EMT_ML.before_diagnostic_fixes/Control Unit/Driver/Pedal /Auto ==
  1-D Lookup Table1 : Lookup_n-D  NumberOfTableDimensions=1  BreakpointsForDimension1=[-10 -3 -2 -1 0 1 2 10]  Table=[-10 -1 0 0.2 1 2 5 10]  RndMeth=Simplest
  1-D Lookup Table2 : Lookup_n-D  NumberOfTableDimensions=1  BreakpointsForDimension1=[-10 -2 -1 -0.5 0 0.5 1 2 10]  Table=[-1 -0.1 -0.01 -0.001 0 0.001 0.01 0.1 1]  RndMeth=Simplest
  Add : Sum
  Fcn : Fcn  Expr=sqrt(abs((u(2)*mass*9.8*u(1)/3.6/1000/0.8)/Pe_max))
  Memory{1..4} (4 alike) : Memory
  Mux : Mux  Inputs=2
  Product1 : Product  RndMeth=Zero
  Saturation : Saturate  UpperLimit=10  LowerLimit=-10
  Saturation1 : Saturate  UpperLimit=10  LowerLimit=-10
  Pedal : Outport
  wires:
  [v_com] -> Memory1/1
  [fg_act] -> Memory2/1
  Memory1/1 -> Mux/1
  Memory2/1 -> Mux/2
  Mux/1 -> Fcn/1
  Fcn/1 -> Product1/1
  [dv_act] -> Memory3/1
  Memory3/1 -> Saturation/1
  Saturation/1 -> 1-D Lookup Table1/1
  1-D Lookup Table1/1 -> Product1/2
  Product1/1 -> Add/1
  Add/1 -> Pedal/1
  [dv_act] -> Memory4/1
  Memory4/1 -> Saturation1/1
  Saturation1/1 -> 1-D Lookup Table2/1
  1-D Lookup Table2/1 -> Add/2

== system EMT_ML.before_diagnostic_fixes/Control Unit/Driver/Pedal /Signal Builder ==
  Demux : Demux  Tag=STV Demux  Outputs=1
      settings: DisplayOption=none
  FromWs : FromWorkspace  Tag=STV FromWs  VariableName=tuvar
      SigBuilderData=|
      | common.afterFinalStr = 'Extrapolate'
      | common.sampleTime = 0
      | dataSet.timeRange = [0 10]
      | dataSet.name = 'Group 1'
      | sbobj.Groups.Name = 'Group 1'
      | sbobj.Groups.Signals.Name = 'Signal 1'
      | sbobj.Groups.Signals.XData = [0 4 4 6 6 10]
      | sbobj.Groups.Signals.YData = [0.63 0.63 -0.155 -0.155 -1 -1]
  Signal 1 : Outport  Tag=STV Outport
  wires:
  Demux/1 -> Signal 1/1
  FromWs/1 -> Demux/1

== system EMT_ML.before_diagnostic_fixes/Control Unit/Driver/Pedal /Subsystem ==
  1-D Lookup Table : Lookup_n-D  NumberOfTableDimensions=1  BreakpointsForDimension1=Time  Table=v_cyc  RndMeth=Simplest
  Add : Sum  Inputs=+-
  Clock : Clock
  Forward : Constant  Value=85
  Transfer Fcn1 : TransferFcn  Denominator=[1 1]
  dv : Outport
  tag scope: dv_act=global, v_com=global
  wires:
  Add/1 -> [dv_act], dv/1
  Clock/1 -> 1-D Lookup Table/1
  [v_act] -> Add/2
  Transfer Fcn1/1 -> [v_com], Add/1
  1-D Lookup Table/1 -> Transfer Fcn1/1

== system EMT_ML.before_diagnostic_fixes/Control Unit/Driver/Pedal /Subsystem13 ==
  Subsystem4 : Subsystem
  Subsystem6 : Subsystem
  Out1 : Outport
  Out2 : Outport  Port=2
  Out3 : Outport  Port=3
  Out4 : Outport  Port=4
  Out5 : Outport  Port=5
  Out6 : Outport  Port=6
  Out7 : Outport  Port=7
  Out8 : Outport  Port=8
  wires:
  Subsystem4/4(100) -> Out8/1
  Subsystem4/3(10) -> Out7/1
  Subsystem4/2(0.01) -> Out6/1
  Subsystem4/1(0.1) -> Out5/1
  Subsystem6/4(4) -> Out4/1
  Subsystem6/3(3) -> Out3/1
  Subsystem6/2(2) -> Out2/1
  Subsystem6/1(1) -> Out1/1

== system EMT_ML.before_diagnostic_fixes/Control Unit/Driver/Pedal /Subsystem5 ==
  Add : Inport
  Sub : Inport  Port=2
  0.1 : Inport  Port=3
  10 : Inport  Port=4
  0.2 : InportShadow  Port=3
  1 : InportShadow  Port=4
  Add1 : Sum  Inputs=++-
  Memory1 : Memory
  Subsystem : Subsystem
  Subsystem1 : Subsystem
  Pedal : Outport
  wires:
  Add1/1 -> Pedal/1, Memory1/1
  Memory1/1 -> Add1/1
  Subsystem1/1(pedal--) -> Add1/3
  Subsystem/1(pedal++) -> Add1/2
  0.1/1 -> Subsystem/1(0.1)
  Add/1 -> Subsystem/2(Add)
  10/1 -> Subsystem/3(10)
  Sub/1 -> Subsystem1/2(Sub)
  1/1 -> Subsystem1/3(10)
  0.2/1 -> Subsystem1/1(0.1)

== system EMT_ML.before_diagnostic_fixes/Control Unit/Driver/Wheel Angle/Subsystem1 ==
  Subsystem4 : Subsystem
  Subsystem6 : Subsystem
  Out1 : Outport
  Out2 : Outport  Port=2
  Out3 : Outport  Port=3
  Out4 : Outport  Port=4
  Out5 : Outport  Port=5
  Out6 : Outport  Port=6
  Out7 : Outport  Port=7
  Out8 : Outport  Port=8
  wires:
  Subsystem4/4(100) -> Out8/1
  Subsystem4/3(10) -> Out7/1
  Subsystem4/2(0.01) -> Out6/1
  Subsystem4/1(0.1) -> Out5/1
  Subsystem6/4(4) -> Out4/1
  Subsystem6/3(3) -> Out3/1
  Subsystem6/2(2) -> Out2/1
  Subsystem6/1(1) -> Out1/1

== system EMT_ML.before_diagnostic_fixes/Control Unit/Driver/Wheel Angle/Subsystem2 ==
  Add : Inport
  Sub : Inport  Port=2
  0.1 : Inport  Port=3
  10 : Inport  Port=4
  0.2 : InportShadow  Port=3
  1 : InportShadow  Port=4
  Add1 : Sum  Inputs=++-
  Memory1 : Memory
  Saturation : Saturate  UpperLimit=15  LowerLimit=-15
  Subsystem : Subsystem
  Subsystem1 : Subsystem
  Transfer Fcn1 : TransferFcn  Denominator=[0.02 1]
  wheel : Outport
  wires:
  Add1/1 -> Memory1/1, Saturation/1
  Memory1/1 -> Add1/1
  Subsystem1/1(wheel--) -> Add1/3
  Saturation/1 -> Transfer Fcn1/1
  Subsystem/1(wheel++) -> Add1/2
  0.1/1 -> Subsystem/1(0.1)
  Add/1 -> Subsystem/2(Add)
  10/1 -> Subsystem/3(10)
  Sub/1 -> Subsystem1/2(Sub)
  1/1 -> Subsystem1/3(10)
  0.2/1 -> Subsystem1/1(0.1)
  Transfer Fcn1/1 -> wheel/1

== system EMT_ML.before_diagnostic_fixes/Front Gear/C0/C0/Slip Sensor ==
  Abs : Abs  SaturateOnIntegerOverflow=off
  Ideal Rotational Motion Sensor : fl_lib/Mechanical/Mechanical Sensors/Ideal Rotational Motion Sensor  reference=foundation.enum.MeasurementReference.difference  acceleration_port=false  velocity_port=true  position_port=true  wrap_angle=false  offset=0 rad
  PS-Simulink Converter : nesl_utility/PS-Simulink Converter  PhysicalDomain=network_engine_domain  SubClassName=ps_output  LeftPortType=input  RightPortType=output  PseudoPeriodic=off  Frequencies=[]  VectorFormat=1-D array  Unit=1  AffineConversion=off
  Tire Radius2 : Gain  Gain=30/pi
  In : PMIOPort  Side=Left
  Out : PMIOPort  Port=2  Side=Right
  r/min : Outport
  wires:
  PS-Simulink Converter/1 -> Tire Radius2/1
  Tire Radius2/1 -> Abs/1
  Abs/1 -> r/min/1
  connections:
  PS-Simulink Converter/LConn1 -- Ideal Rotational Motion Sensor/RConn2
  Out/RConn1 -- Ideal Rotational Motion Sensor/RConn1
  In/RConn1 -- Ideal Rotational Motion Sensor/LConn1

== system EMT_ML.before_diagnostic_fixes/Front Gear/C0/Power/Speed Sensor ==
  Ideal Rotational Motion Sensor : fl_lib/Mechanical/Mechanical Sensors/Ideal Rotational Motion Sensor  reference=foundation.enum.MeasurementReference.difference  acceleration_port=false  velocity_port=true  position_port=true  wrap_angle=false  offset=0 rad
  PS-Simulink Converter : nesl_utility/PS-Simulink Converter  PhysicalDomain=network_engine_domain  SubClassName=ps_output  LeftPortType=input  RightPortType=output  PseudoPeriodic=off  Frequencies=[]  VectorFormat=1-D array  Unit=rad/s  AffineConversion=off
  Reference : fl_lib/Mechanical/Rotational Elements/Mechanical Rotational Reference
  Tire Radius2 : Gain  Gain=30/pi
  shaft : PMIOPort  Side=Left
  r/min : Outport
  wires:
  PS-Simulink Converter/1 -> Tire Radius2/1
  Tire Radius2/1 -> r/min/1
  connections:
  PS-Simulink Converter/LConn1 -- Ideal Rotational Motion Sensor/RConn2
  Reference/LConn1 -- Ideal Rotational Motion Sensor/RConn1
  shaft/RConn1 -- Ideal Rotational Motion Sensor/LConn1

== system EMT_ML.before_diagnostic_fixes/Front Gear/C0/Power/Torque Sensor ==
  Ideal Torque Sensor : fl_lib/Mechanical/Mechanical Sensors/Ideal Torque Sensor
  PS-Simulink Converter : nesl_utility/PS-Simulink Converter  PhysicalDomain=network_engine_domain  SubClassName=ps_output  LeftPortType=input  RightPortType=output  PseudoPeriodic=off  Frequencies=[]  VectorFormat=1-D array  Unit=1  AffineConversion=off
  In : PMIOPort  Side=Left
  Out : PMIOPort  Port=2  Side=Right
  Nm : Outport
  wires:
  PS-Simulink Converter/1 -> Nm/1
  connections:
  Ideal Torque Sensor/RConn1 -- Out/RConn1
  In/RConn1 -- Ideal Torque Sensor/LConn1
  PS-Simulink Converter/LConn1 -- Ideal Torque Sensor/RConn2

== system EMT_ML.before_diagnostic_fixes/Front Gear/C0/Power1/Speed Sensor ==
  Ideal Rotational Motion Sensor : fl_lib/Mechanical/Mechanical Sensors/Ideal Rotational Motion Sensor  reference=foundation.enum.MeasurementReference.difference  acceleration_port=false  velocity_port=true  position_port=true  wrap_angle=false  offset=0 rad
  PS-Simulink Converter : nesl_utility/PS-Simulink Converter  PhysicalDomain=network_engine_domain  SubClassName=ps_output  LeftPortType=input  RightPortType=output  PseudoPeriodic=off  Frequencies=[]  VectorFormat=1-D array  Unit=rad/s  AffineConversion=off
  Reference : fl_lib/Mechanical/Rotational Elements/Mechanical Rotational Reference
  Tire Radius2 : Gain  Gain=30/pi
  shaft : PMIOPort  Side=Left
  r/min : Outport
  wires:
  Tire Radius2/1 -> r/min/1
  PS-Simulink Converter/1 -> Tire Radius2/1
  connections:
  shaft/RConn1 -- Ideal Rotational Motion Sensor/LConn1
  Reference/LConn1 -- Ideal Rotational Motion Sensor/RConn1
  PS-Simulink Converter/LConn1 -- Ideal Rotational Motion Sensor/RConn2

== system EMT_ML.before_diagnostic_fixes/Front Gear/C0/Power1/Torque Sensor ==
  Ideal Torque Sensor : fl_lib/Mechanical/Mechanical Sensors/Ideal Torque Sensor
  PS-Simulink Converter : nesl_utility/PS-Simulink Converter  PhysicalDomain=network_engine_domain  SubClassName=ps_output  LeftPortType=input  RightPortType=output  PseudoPeriodic=off  Frequencies=[]  VectorFormat=1-D array  Unit=1  AffineConversion=off
  In : PMIOPort  Side=Left
  Out : PMIOPort  Port=2  Side=Right
  Nm : Outport
  wires:
  PS-Simulink Converter/1 -> Nm/1
  connections:
  PS-Simulink Converter/LConn1 -- Ideal Torque Sensor/RConn2
  In/RConn1 -- Ideal Torque Sensor/LConn1
  Ideal Torque Sensor/RConn1 -- Out/RConn1

== system EMT_ML.before_diagnostic_fixes/Power Coupler /C1/C2/Slip Sensor ==
  Abs : Abs  SaturateOnIntegerOverflow=off
  Ideal Rotational Motion Sensor : fl_lib/Mechanical/Mechanical Sensors/Ideal Rotational Motion Sensor  reference=foundation.enum.MeasurementReference.difference  acceleration_port=false  velocity_port=true  position_port=true  wrap_angle=false  offset=0 rad
  PS-Simulink Converter : nesl_utility/PS-Simulink Converter  PhysicalDomain=network_engine_domain  SubClassName=ps_output  LeftPortType=input  RightPortType=output  PseudoPeriodic=off  Frequencies=[]  VectorFormat=1-D array  Unit=1  AffineConversion=off
  Tire Radius2 : Gain  Gain=30/pi
  In : PMIOPort  Side=Left
  Out : PMIOPort  Port=2  Side=Right
  r/min : Outport
  wires:
  Abs/1 -> r/min/1
  Tire Radius2/1 -> Abs/1
  PS-Simulink Converter/1 -> Tire Radius2/1
  connections:
  In/RConn1 -- Ideal Rotational Motion Sensor/LConn1
  Out/RConn1 -- Ideal Rotational Motion Sensor/RConn1
  PS-Simulink Converter/LConn1 -- Ideal Rotational Motion Sensor/RConn2

== system EMT_ML.before_diagnostic_fixes/Power Coupler /C1/Power/Speed Sensor ==
  Ideal Rotational Motion Sensor : fl_lib/Mechanical/Mechanical Sensors/Ideal Rotational Motion Sensor  reference=foundation.enum.MeasurementReference.difference  acceleration_port=false  velocity_port=true  position_port=true  wrap_angle=false  offset=0 rad
  PS-Simulink Converter : nesl_utility/PS-Simulink Converter  PhysicalDomain=network_engine_domain  SubClassName=ps_output  LeftPortType=input  RightPortType=output  PseudoPeriodic=off  Frequencies=[]  VectorFormat=1-D array  Unit=rad/s  AffineConversion=off
  Reference : fl_lib/Mechanical/Rotational Elements/Mechanical Rotational Reference
  Tire Radius2 : Gain  Gain=30/pi
  shaft : PMIOPort  Side=Left
  r/min : Outport
  wires:
  Tire Radius2/1 -> r/min/1
  PS-Simulink Converter/1 -> Tire Radius2/1
  connections:
  shaft/RConn1 -- Ideal Rotational Motion Sensor/LConn1
  Reference/LConn1 -- Ideal Rotational Motion Sensor/RConn1
  PS-Simulink Converter/LConn1 -- Ideal Rotational Motion Sensor/RConn2

== system EMT_ML.before_diagnostic_fixes/Power Coupler /C1/Power/Torque Sensor ==
  Ideal Torque Sensor : fl_lib/Mechanical/Mechanical Sensors/Ideal Torque Sensor
  PS-Simulink Converter : nesl_utility/PS-Simulink Converter  PhysicalDomain=network_engine_domain  SubClassName=ps_output  LeftPortType=input  RightPortType=output  PseudoPeriodic=off  Frequencies=[]  VectorFormat=1-D array  Unit=1  AffineConversion=off
  In : PMIOPort  Side=Left
  Out : PMIOPort  Port=2  Side=Right
  Nm : Outport
  wires:
  PS-Simulink Converter/1 -> Nm/1
  connections:
  PS-Simulink Converter/LConn1 -- Ideal Torque Sensor/RConn2
  In/RConn1 -- Ideal Torque Sensor/LConn1
  Ideal Torque Sensor/RConn1 -- Out/RConn1

== system EMT_ML.before_diagnostic_fixes/Power Coupler /C1/Power1/Speed Sensor ==
  Ideal Rotational Motion Sensor : fl_lib/Mechanical/Mechanical Sensors/Ideal Rotational Motion Sensor  reference=foundation.enum.MeasurementReference.difference  acceleration_port=false  velocity_port=true  position_port=true  wrap_angle=false  offset=0 rad
  PS-Simulink Converter : nesl_utility/PS-Simulink Converter  PhysicalDomain=network_engine_domain  SubClassName=ps_output  LeftPortType=input  RightPortType=output  PseudoPeriodic=off  Frequencies=[]  VectorFormat=1-D array  Unit=rad/s  AffineConversion=off
  Reference : fl_lib/Mechanical/Rotational Elements/Mechanical Rotational Reference
  Tire Radius2 : Gain  Gain=30/pi
  shaft : PMIOPort  Side=Left
  r/min : Outport
  wires:
  PS-Simulink Converter/1 -> Tire Radius2/1
  Tire Radius2/1 -> r/min/1
  connections:
  PS-Simulink Converter/LConn1 -- Ideal Rotational Motion Sensor/RConn2
  Reference/LConn1 -- Ideal Rotational Motion Sensor/RConn1
  shaft/RConn1 -- Ideal Rotational Motion Sensor/LConn1

== system EMT_ML.before_diagnostic_fixes/Power Coupler /C1/Power1/Torque Sensor ==
  Ideal Torque Sensor : fl_lib/Mechanical/Mechanical Sensors/Ideal Torque Sensor
  PS-Simulink Converter : nesl_utility/PS-Simulink Converter  PhysicalDomain=network_engine_domain  SubClassName=ps_output  LeftPortType=input  RightPortType=output  PseudoPeriodic=off  Frequencies=[]  VectorFormat=1-D array  Unit=1  AffineConversion=off
  In : PMIOPort  Side=Left
  Out : PMIOPort  Port=2  Side=Right
  Nm : Outport
  wires:
  PS-Simulink Converter/1 -> Nm/1
  connections:
  Ideal Torque Sensor/RConn1 -- Out/RConn1
  In/RConn1 -- Ideal Torque Sensor/LConn1
  PS-Simulink Converter/LConn1 -- Ideal Torque Sensor/RConn2

== system EMT_ML.before_diagnostic_fixes/Power Coupler /Z1/Z/Power ==
  Gain1 : Gain  Gain=1/9549
  Product3 : Product  RndMeth=Zero
  Speed Sensor : Subsystem  mask(Speed Sensor){}
      mask help: The speed unit is r/min.
  Torque Sensor : Subsystem  mask(Torque Sensor){}
      mask help: The torque unit is Nm.
  In : PMIOPort  Side=Left
  Out : PMIOPort  Port=2  Side=Right
  kW : Outport
  wires:
  Product3/1 -> kW/1
  Gain1/1 -> Product3/1
  Torque Sensor/1(Nm) -> Gain1/1
  Speed Sensor/1(r/min) -> Product3/2
  connections:
  In/RConn1 -- Torque Sensor/LConn1
  Torque Sensor/RConn1 -- Out/RConn1 -- Speed Sensor/LConn1

== system EMT_ML.before_diagnostic_fixes/Power Coupler /Z1/Z/Power1 ==
  Gain1 : Gain  Gain=1/9549
  Product3 : Product  RndMeth=Zero
  Speed Sensor : Subsystem  mask(Speed Sensor){}
      mask help: The speed unit is r/min.
  Torque Sensor : Subsystem  mask(Torque Sensor){}
      mask help: The torque unit is Nm.
  In : PMIOPort  Side=Left
  Out : PMIOPort  Port=2  Side=Right
  kW : Outport
  wires:
  Speed Sensor/1(r/min) -> Product3/2
  Torque Sensor/1(Nm) -> Gain1/1
  Gain1/1 -> Product3/1
  Product3/1 -> kW/1
  connections:
  Speed Sensor/LConn1 -- Out/RConn1 -- Torque Sensor/RConn1
  In/RConn1 -- Torque Sensor/LConn1

== system EMT_ML.before_diagnostic_fixes/Power Coupler /Z1/Z/Z1 ==
  Press : Inport
  Simulink-PS Converter : nesl_utility/Simulink-PS Converter  PhysicalDomain=network_engine_domain  SubClassName=ps_input  LeftPortType=input  RightPortType=output  PseudoPeriodic=off  Frequencies=[]  NoiseDistribution=none  NoiseParameters=[]  Unit=Pa  AffineConversion=off  FilteringAndDerivatives=filter  SimscapeFilterOrder=1  InputFilterTimeConstant=.001  UdotUserProvided=1
  Slip Sensor : Subsystem  mask(Slip Sensor){}
      mask help: The speed unit is r/min.
  Tire Radius2 : Gain  Gain=2500000
  Z1 : sdl_lib/Clutches/Disc Friction Clutch  geometry_model=2  r_eff=130 mm  d_o=207*2 mm  d_i=174.25*2 mm  nS=12  piston_area=0.0528 m^2  unidirectional=0  friction_model=1  mu_w_vector=[ 0 0.1 0.2 0.3 0.4 0.5 1 2 5 10 100 1000 ] rad/s  temperature_TLU=[280.0, 300.0, 320.0] K  mu_static=0.10  mu_static_vector=[0.4, 0.38, 0.36]  mu_coulomb=0.06  mu_coulomb_vector=[ 0.29 0.28 0.26 0.22 0.21 0.2 0.2 0.19 0.19 0.19 0.19 0.19 ]  mu_coulomb_temp_vector=[0.3, 0.28, 0.25]  mu_coulomb_matrix=[0.34, 0.32, 0.3; 0.3, 0.28, 0.25; 0.25, 0.2, 0.15]  mu_interp_method=1  mu_extrap_method=1  d_f=0.6  w_tol=0.001 rad/s  pressure_min=1930 Pa  mu_visc=0.1580 N*m/(rad/s)  initial_state_locked=0  thermal_mass=25 kJ/K  T_init=300 K
      settings: InternalSimscapePortConfiguration="{\"Bottom\":[],\"Left\":[{\"id\":\"P\",\"label\":\"P\",\"type\":\"input\"},{\"id\":\"B\",\"label\":\"B\",\"type\":\"foundation.mechanical.rotational.rotational\"}],\"Right\":[{\"id\":\"F\",\"label\":\"F\",\"type\":\"foundation.mechanical.rotational.rotational\"}],\"Top\":[]}"
  In : PMIOPort  Side=Left
  Out : PMIOPort  Port=2  Side=Right
  r/min : Outport
  wires:
  Slip Sensor/1(r/min) -> r/min/1
  Press/1 -> Tire Radius2/1
  Tire Radius2/1 -> Simulink-PS Converter/1
  connections:
  Slip Sensor/RConn1 -- Out/RConn1 -- Z1/RConn1
  Slip Sensor/LConn1 -- Z1/LConn2 -- In/RConn1
  Simulink-PS Converter/RConn1 -- Z1/LConn1

== system EMT_ML.before_diagnostic_fixes/Power Coupler /Z2/Z/Power ==
  Gain1 : Gain  Gain=1/9549
  Product3 : Product  RndMeth=Zero
  Speed Sensor : Subsystem  mask(Speed Sensor){}
      mask help: The speed unit is r/min.
  Torque Sensor : Subsystem  mask(Torque Sensor){}
      mask help: The torque unit is Nm.
  In : PMIOPort  Side=Left
  Out : PMIOPort  Port=2  Side=Right
  kW : Outport
  wires:
  Product3/1 -> kW/1
  Gain1/1 -> Product3/1
  Torque Sensor/1(Nm) -> Gain1/1
  Speed Sensor/1(r/min) -> Product3/2
  connections:
  In/RConn1 -- Torque Sensor/LConn1
  Torque Sensor/RConn1 -- Out/RConn1 -- Speed Sensor/LConn1

== system EMT_ML.before_diagnostic_fixes/Power Coupler /Z2/Z/Power1 ==
  Gain1 : Gain  Gain=1/9549
  Product3 : Product  RndMeth=Zero
  Speed Sensor : Subsystem  mask(Speed Sensor){}
      mask help: The speed unit is r/min.
  Torque Sensor : Subsystem  mask(Torque Sensor){}
      mask help: The torque unit is Nm.
  In : PMIOPort  Side=Left
  Out : PMIOPort  Port=2  Side=Right
  kW : Outport
  wires:
  Speed Sensor/1(r/min) -> Product3/2
  Torque Sensor/1(Nm) -> Gain1/1
  Gain1/1 -> Product3/1
  Product3/1 -> kW/1
  connections:
  Speed Sensor/LConn1 -- Out/RConn1 -- Torque Sensor/RConn1
  In/RConn1 -- Torque Sensor/LConn1
